simulink model "lead_lad"  (R2025b)
settings: Solver=VariableStepAuto  StartTime=0.0  StopTime=10.0  RelTol=1e-3
settings Model: Creator=alosw  LastModifiedBy=alosw

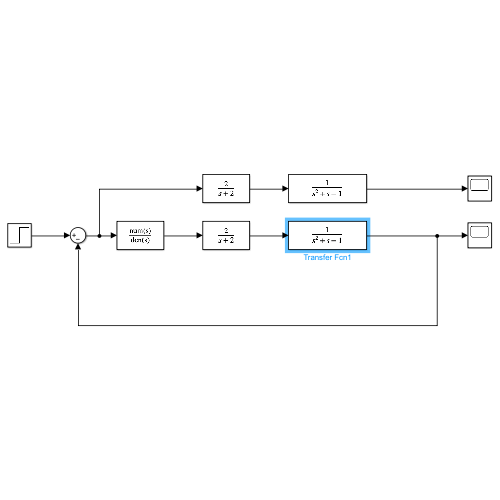
[thumbnail: Simulink's stored preview of the top-level diagram]
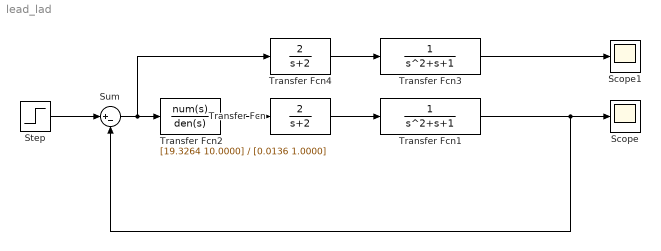
== system lead_lad ==
  Scope : Scope
      settings: ActiveDisplayYMinimum=-346.50286651409021  ActiveDisplayYMaximum=541.89230226935206
  Scope1 : Scope
      settings: ActiveDisplayYMinimum=-1.1007408750256562  ActiveDisplayYMaximum=1.3445836841231615
  Step : Step  SampleTime=0
  Sum : Sum  Inputs=|+-
  Transfer Fcn : TransferFcn  Numerator=[2]  Denominator=[1 2]
  Transfer Fcn1 : TransferFcn  Denominator=[1 1 1]
  Transfer Fcn2 : TransferFcn  Numerator=[19.3264 10.0000]  Denominator=[0.0136 1.0000]
  Transfer Fcn3 : TransferFcn  Denominator=[1 1 1]
  Transfer Fcn4 : TransferFcn  Numerator=[2]  Denominator=[1 2]
  wires:
  Transfer Fcn/1 -> Transfer Fcn1/1
  Sum/1 -> Transfer Fcn4/1, Transfer Fcn2/1
  Step/1 -> Sum/1
  Transfer Fcn4/1 -> Transfer Fcn3/1
  Transfer Fcn3/1 -> Scope1/1
  Transfer Fcn1/1 -> Scope/1, Sum/2
  Transfer Fcn2/1 -> Transfer Fcn/1
